simulink model "heli_q8_lab4_2020b"  (R2020b)
settings: Solver=ode1  StartTime=0.0  StopTime=inf  FixedStep=0.002  RelTol=1e-3  EnableMultiTasking=on
PostLoadFcn:
  | qc_set_target_type(getConfigSet(bdroot, 'QUARC Default Target Configuration'));
values from neighbouring files (symbols this model uses):
  Ad = sysd.A    [init_heli_3_10_part_4.m]    (also in tune_qw_offline.m = sd.A)
  Bd = sysd.B    [init_heli_3_10_part_4.m]    (also in tune_qw_offline.m = sd.B)
  Cd = sysd.C    [init_heli_3_10_part_4.m]    (also in tune_qw_offline.m = sd.C)
  elev_const = 0.53    [init_heli_3_10_part_4.m]
  F_2 = [K_2(1,1) K_2(1,3) ... (first row only)    [init_heli_3_10_part_4.m]
  gyro_bias = [0.0392850152533 -0.00867648252983 0.000660862987064]    [imu_bias.mat]    (also in update_imu_bias.m = mean(d(idx,13:15))')
  imu_bias = [-0.0918732538603 0 0.0496947738021 0 0]    [imu_bias.mat]    (also in update_imu_bias.m = imu_bias + mean(d(idx,2:6) - d(idx,8:12))')
  Joystick_gain_x = 1    [init_heli_3_10_part_4.m]
  Joystick_gain_y = -1    [init_heli_3_10_part_4.m]
  K_2 = lqr(A_lqr,B_lqr,Q_lqr, R_lqr)    [init_heli_3_10_part_4.m]
  P0 = blkdiag(P0, 0.02^2*eye(3))    [init_heli_3_10_part_4.m]
  Qd = Qd6    [init_heli_3_10_part_4.m]    (also in tune_qw_offline.m = blkdiag(Qd, 1e-11*eye(3)))
  Rd = [0.000112260066924 4.65584239908e-05 -7.15809020323e-05 -6.37518998984e-05 -2.81466202083e-06 4.65584239908e-05 0.000458002814453 2.17937662307e-05 -6.23292915171e-05 -4.71096272763e-06 -7.15809020323e-05 2.17937662307e-05 ... (25 elements, 5x5)]    [Rd.mat]    (also in analyze_noise.m = Rd_fly; estimate_Rd.m = cov(noise))
  V_s_0 = 7.77    [init_heli_3_10_part_4.m]
  x0 = [x0; 0; 0; 0]    [init_heli_3_10_part_4.m]
undefined symbols (not defined in the file or in its folder): HIL, qc_get_step_size, sigbuilder_block
libraries: quarc_library x9
settings Model: SimulationMode=external  ExtModeTrigDuration=50000  Creator=Rchan  LastModifiedBy=saavim
settings SolverCC: PositivePriorityOrder=on
settings DataIOCC: LimitDataPoints=on  SaveFormat=Array  SignalLoggingSaveFormat=ModelDataLogs  ReturnWorkspaceOutputs=off
settings OptimizationCC: ExpressionDepthLimit=2147483647  InitFltsAndDblsToZero=on  LifeSpan=inf
settings DebuggingCC: SaveWithParameterizedLinksMsg=none  UnderspecifiedInitializationDetection=Classic  MergeDetectMultiDrivingBlocksExec=none  SolverPrmCheckMsg=warning  MultiTaskDSMMsg=warning  MultiTaskCondExecSysMsg=none  FcnCallInpInsideContextMsg=warning  AllowSymbolicDim=off  StateNameClashWarn=warning  SFUnexpectedBacktrackingDiag=warning  SFNoUnconditionalDefaultTransitionDiag=warning  SFExecutionAtInitializationDiag=none  ArithmeticOperatorsInVariantConditions=warning
settings HardwareCC: ProdBitPerPointer=32  ProdBitPerSizeT=32  ProdBitPerPtrDiffT=32  ProdLargestAtomicFloat=None  ProdIntDivRoundTo=Undefined  ProdEndianess=Unspecified  ProdWordSize=32  ProdHWDeviceType=32-bit Generic
settings ModelReferenceCC: PropagateSignalLabelsOutOfModel=off
settings SFSimCC: SimUseLocalCustomCode=off  CustomCodeUndefinedFunction=UseInterfaceOnly
settings RTWCC: Description=QUARC Win64 Target  SystemTargetFile=quarc_win64.tlc  TemplateMakefile=quarc_default_tmf  RTWUseLocalCustomCode=off
settings CodeAppCC: StateflowObjectComments=on
settings STFCustomTargetCC: MatFileLogging=on
settings GRTTargetCC: TargetLangStandard=C89/C90 (ANSI)  ParMdlRefBuildCompliant=off  CompOptLevelCompliant=off  CombineOutputUpdateFcns=off  GRTInterface=on  UseToolchainInfoCompliant=off  ExtMode=on  ExtModeMexFile=quarc_comm
settings ConfigComp: CovMetricSettings=de  CovSaveCumulativeToWorkspaceVar=on  CovSaveSingleToWorkspaceVar=on  CovExternalEMLEnable=off  CovSFcnEnable=off

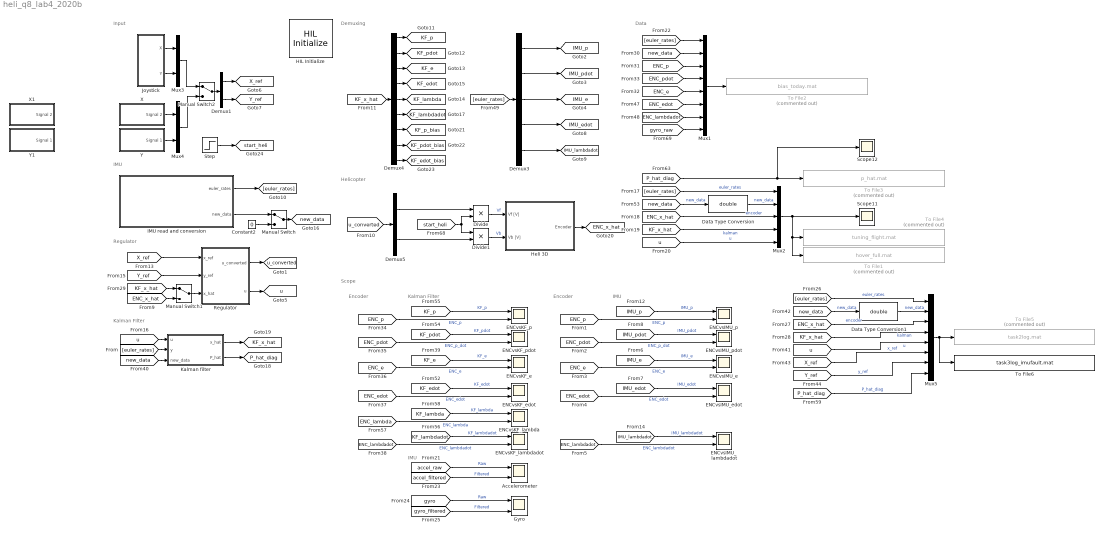
== system heli_q8_lab4_2020b ==
  note: Data
  note: Scope
  note: Helicopter
  note: Regulator
  note: IMU
  note: Kalman FIlter
  note: Input
  note: Demuxing
  note: Encoder
  note: Kalman Filter
  note: IMU
  note: Encoder
  note: IMU
  Accelerometer : Scope  NumInputPorts=2
  Constant2 : Constant  Value=0
  Data Type Conversion : DataTypeConversion  OutDataTypeStr=double  LockScale=on
  Data Type Conversion1 : DataTypeConversion  OutDataTypeStr=double  LockScale=on
  Demux1 : Demux  Outputs=2
  Demux3 : Demux  Outputs=5
  Demux4 : Demux  Outputs=9
  Demux5 : Demux  Outputs=2
  Divide : Product  Inputs=**
  Divide1 : Product  Inputs=**
  ENCvsIMU_e : Scope  NumInputPorts=2
  ENCvsIMU_edot : Scope  NumInputPorts=2
  ENCvsIMU_lambdadot : Scope  NumInputPorts=2
  ENCvsIMU_p : Scope  NumInputPorts=2
  ENCvsIMU_pdot : Scope  NumInputPorts=2
  ENCvsKF_e : Scope  NumInputPorts=2
  ENCvsKF_edot : Scope  NumInputPorts=2
  ENCvsKF_lambda : Scope  NumInputPorts=2
  ENCvsKF_lambdadot : Scope  NumInputPorts=2
  ENCvsKF_p : Scope  NumInputPorts=2
  ENCvsKF_pdot : Scope  NumInputPorts=2
  Gyro : Scope  NumInputPorts=2
  HIL Initialize : quarc_library/Data Acquisition/Generic/Configuration/HIL Initialize  Priority=-99  object_name=HIL-1  board_type=q8_usb  board_number=0  board_options=update_rate=normal;decimation=1  exclusive=off  active=off  hardware_clocks=[0:2]  clock_modes=[]  initial_clock_frequencies=[]  set_clock_params_at_start=off  set_clock_params_at_switch_in=off  set_clock_frequencies_at_start=off  set_clock_frequencies_at_switch_in=off  analog_input_channels=[0:7]  analog_input_configurations=[]  analog_input_maximums=10  analog_input_minimums=-10  set_analog_input_params_at_start=on  set_analog_input_params_at_switch_in=off  analog_output_channels=[0:7]  analog_output_maximums=10  analog_output_minimums=-10  initial_analog_outputs=[0]  final_analog_outputs=[0]  watchdog_analog_outputs=0  set_analog_output_params_at_start=on  set_analog_output_params_at_switch_in=off  set_analog_outputs_at_start=on  set_analog_outputs_at_switch_in=off  set_analog_outputs_at_terminate=on  set_analog_outputs_at_switch_out=off  set_analog_outputs_on_watchdog=off  digital_input_channels=[]  digital_output_channels=[]  digital_output_configuration=[]  initial_digital_outputs=[1]  final_digital_outputs=[1]  watchdog_digital_outputs=[1]  set_digital_output_params_at_start=off  set_digital_output_params_at_switch_in=off  set_digital_outputs_at_start=on  set_digital_outputs_at_switch_in=off  set_digital_outputs_at_terminate=on  set_digital_outputs_at_switch_out=off  set_digital_outputs_on_watchdog=off  encoder_channels=[0:7]  quadrature=[4]  encoder_filter_frequency=[]  initial_encoder_counts=[0]  set_encoder_params_at_start=on  set_encoder_params_at_switch_in=off  set_encoder_counts_at_start=on  set_encoder_counts_at_switch_in=off  pwm_channels=[0:7]  pwm_modes=0  pwm_frequency=99.532799999999995e6/4095  pwm_configuration=[0]  pwm_alignment=[0]  pwm_polarity=[1]  pwm_leading_deadband=[0]  pwm_trailing_deadband=[0]  initial_pwm_outputs=[0]  final_pwm_outputs=[0]  watchdog_pwm_outputs=[0]  set_pwm_params_at_start=on  set_pwm_params_at_switch_in=off  set_pwm_outputs_at_start=on  set_pwm_outputs_at_switch_in=off  set_pwm_outputs_at_terminate=on  set_pwm_outputs_at_switch_out=off  set_pwm_outputs_on_watchdog=off  other_output_channels=[]  initial_other_outputs=[]  final_other_outputs=[]  watchdog_other_outputs=[]  set_other_outputs_at_start=off  set_other_outputs_at_switch_in=off  set_other_outputs_at_terminate=off  set_other_outputs_at_switch_out=off  set_other_outputs_on_watchdog=off
  Heli 3D : Subsystem
  IMU read and conversion : Subsystem
  Joystick : Subsystem
  Kalman filter : Subsystem
  Manual Switch : ManualSwitch
  Manual Switch1 : ManualSwitch
  Manual Switch2 : ManualSwitch
  Mux1 : Mux  Inputs=8
  Mux2 : Mux  Inputs=5
  Mux3 : Mux  Inputs=2
  Mux4 : Mux  Inputs=2
  Mux5 : Mux  Inputs=8
  Regulator : Subsystem
  Scope11 : Scope
  Scope12 : Scope
  Step : Step  Time=3  SampleTime=0
  To File1 : ToFile  Commented=on  Filename=hover_full.mat  MatrixName=hover_full  SampleTime=0.002
  To File2 : ToFile  Commented=on  Filename=bias_today.mat  MatrixName=bias_today
  To File3 : ToFile  Commented=on  Filename=p_hat.mat  MatrixName=p_hat  SampleTime=0.002
  To File4 : ToFile  Commented=on  Filename=tuning_flight.mat  MatrixName=tuning_flight  SampleTime=0.002
  To File5 : ToFile  Commented=on  Filename=task2log.mat  MatrixName=task2log  SampleTime=0.002
  To File6 : ToFile  Filename=task3log_imufault.mat  MatrixName=task3log_imufault  SampleTime=0.002
  X : Subsystem  Tag=STV Subsys  LoadFcn=sigbuilder_block('load');  StartFcn=sigbuilder_block('start');  StopFcn=sigbuilder_block('stop');  ClipboardFcn=sigbuilder_block('clipboard');  mask(Sigbuilder block){tuvar=[0:10]}
      mask help: Simulink:masks:SigbuilderBlock_MD
      mask init:
      | if ~strcmp(get_param(bdroot(gcbh),'SimulationStatus'),'stopped') tuvar = sigbuilder_block('maskInit'); end
      settings: CopyFcn=sigbuilder_block('copy');  DeleteFcn=sigbuilder_block('delete');  ModelCloseFcn=sigbuilder_block('modelClose');  PreSaveFcn=sigbuilder_block('preSave');  PauseFcn=sigbuilder_block('pause');  ContinueFcn=sigbuilder_block('continue');  NameChangeFcn=sigbuilder_block('namechange');  OpenFcn=sigbuilder_block('open',[0 172 1440 619 ]);  CloseFcn=sigbuilder_block('close');
      mask Display: plot(0, 0, 100, 100,[2, 2, 32, 32, 2], [68, 8, 8, 68, 68],[32, 2], [38, 38], [32, 19, 2],[53, 60, 44], [32, 17, 17, 2],[16, 16, 31, 31]);txt = getActiveGroup(gcbh);text(2, 100, txt,'verticalAlignment', 'top');
  X1 : Subsystem  Tag=STV Subsys  LoadFcn=sigbuilder_block('load');  StartFcn=sigbuilder_block('start');  StopFcn=sigbuilder_block('stop');  ClipboardFcn=sigbuilder_block('clipboard');  mask(Sigbuilder block){tuvar=[0:10]}
      mask help: Simulink:masks:SigbuilderBlock_MD
      mask init:
      | if ~strcmp(get_param(bdroot(gcbh),'SimulationStatus'),'stopped') tuvar = sigbuilder_block('maskInit'); end
      settings: CopyFcn=sigbuilder_block('copy');  DeleteFcn=sigbuilder_block('delete');  ModelCloseFcn=sigbuilder_block('modelClose');  PreSaveFcn=sigbuilder_block('preSave');  PauseFcn=sigbuilder_block('pause');  ContinueFcn=sigbuilder_block('continue');  NameChangeFcn=sigbuilder_block('namechange');  OpenFcn=sigbuilder_block('open',[0 172 1440 619 ]);  CloseFcn=sigbuilder_block('close');
      mask Display: plot(0, 0, 100, 100,[2, 2, 32, 32, 2], [68, 8, 8, 68, 68],[32, 2], [38, 38], [32, 19, 2],[53, 60, 44], [32, 17, 17, 2],[16, 16, 31, 31]);txt = getActiveGroup(gcbh);text(2, 100, txt,'verticalAlignment', 'top');
  Y : Subsystem  Tag=STV Subsys  LoadFcn=sigbuilder_block('load');  StartFcn=sigbuilder_block('start');  StopFcn=sigbuilder_block('stop');  ClipboardFcn=sigbuilder_block('clipboard');  mask(Sigbuilder block){tuvar=[0:10]}
      mask help: Simulink:masks:SigbuilderBlock_MD
      mask init:
      | if ~strcmp(get_param(bdroot(gcbh),'SimulationStatus'),'stopped') tuvar = sigbuilder_block('maskInit'); end
      settings: CopyFcn=sigbuilder_block('copy');  DeleteFcn=sigbuilder_block('delete');  ModelCloseFcn=sigbuilder_block('modelClose');  PreSaveFcn=sigbuilder_block('preSave');  PauseFcn=sigbuilder_block('pause');  ContinueFcn=sigbuilder_block('continue');  NameChangeFcn=sigbuilder_block('namechange');  OpenFcn=sigbuilder_block('open',[217.5 306 1336.5 574.5 ]);  CloseFcn=sigbuilder_block('close');
      mask Display: plot(0, 0, 100, 100,[2, 2, 32, 32, 2], [68, 8, 8, 68, 68],[32, 2], [38, 38], [32, 19, 2],[53, 60, 44], [32, 17, 17, 2],[16, 16, 31, 31]);txt = getActiveGroup(gcbh);text(2, 100, txt,'verticalAlignment', 'top');
  Y1 : Subsystem  Tag=STV Subsys  LoadFcn=sigbuilder_block('load');  StartFcn=sigbuilder_block('start');  StopFcn=sigbuilder_block('stop');  ClipboardFcn=sigbuilder_block('clipboard');  mask(Sigbuilder block){tuvar=[0:10]}
      mask help: Simulink:masks:SigbuilderBlock_MD
      mask init:
      | if ~strcmp(get_param(bdroot(gcbh),'SimulationStatus'),'stopped') tuvar = sigbuilder_block('maskInit'); end
      settings: CopyFcn=sigbuilder_block('copy');  DeleteFcn=sigbuilder_block('delete');  ModelCloseFcn=sigbuilder_block('modelClose');  PreSaveFcn=sigbuilder_block('preSave');  PauseFcn=sigbuilder_block('pause');  ContinueFcn=sigbuilder_block('continue');  NameChangeFcn=sigbuilder_block('namechange');  OpenFcn=sigbuilder_block('open',[217.5 306 1336.5 574.5 ]);  CloseFcn=sigbuilder_block('close');
      mask Display: plot(0, 0, 100, 100,[2, 2, 32, 32, 2], [68, 8, 8, 68, 68],[32, 2], [38, 38], [32, 19, 2],[53, 60, 44], [32, 17, 17, 2],[16, 16, 31, 31]);txt = getActiveGroup(gcbh);text(2, 100, txt,'verticalAlignment', 'top');
  tag scope: ENC_x_hat=global, IMU_e=global, IMU_edot=global, IMU_lambdadot=global, IMU_p=global, IMU_pdot=global, KF_e=global, KF_edot=global, KF_edot_bias=global, KF_lambda=global, KF_lambdadot=global, KF_p=global, KF_p_bias=global, KF_pdot=global, KF_pdot_bias=global, KF_x_hat=global, P_hat_diag=global, X_ref=global, Y_ref=global, new_data=global, start_heli=global, u=global, u_converted=global
  wires:
  IMU read and conversion/1(euler_rates) -> [euler_rates]
  Kalman filter/1(x_hat) -> [KF_x_hat]
  Demux4/1 -> [KF_p]
  Demux4/2 -> [KF_pdot]
  Demux4/3 -> [KF_e]
  Demux4/4 -> [KF_edot]
  Demux4/5 -> [KF_lambda]
  [new_data] -> Kalman filter/3(new_data)
  [euler_rates] -> Kalman filter/2(y)
  [new_data] -> Data Type Conversion/1  "new_data"
  Demux4/6 -> [KF_lambdadot]
  Kalman filter/2(P_hat) -> [P_hat_diag]
  Mux2/1 -> To File4/1, To File1/1, Scope11/1
  [P_hat_diag] -> Scope12/1, To File3/1
  IMU read and conversion/2(new_data) -> Manual Switch/1
  Manual Switch/1 -> [new_data]
  Constant2/1 -> Manual Switch/2
  Mux1/1 -> To File2/1
  [euler_rates] -> Mux1/1
  [new_data] -> Mux1/2
  [ENC_p] -> Mux1/3
  [ENC_pdot] -> Mux1/4
  [ENC_e] -> Mux1/5
  [ENC_edot] -> Mux1/6
  [ENC_lambdadot] -> Mux1/7
  [euler_rates] -> Demux3/1
  Demux4/7 -> [KF_p_bias]
  Demux4/8 -> [KF_pdot_bias]
  Demux4/9 -> [KF_edot_bias]
  Step/1 -> [start_heli]
  [start_heli] -> Divide/2, Divide1/1
  [gyro_raw] -> Mux1/8
  Divide/1 -> Heli 3D/1(Vf [V])  "Vf"
  Divide1/1 -> Heli 3D/2(Vb [V])  "Vb"
  Heli 3D/1(Encoder) -> [ENC_x_hat]
  Demux5/2 -> Divide1/2
  Demux5/1 -> Divide/1
  [u_converted] -> Demux5/1
  [KF_x_hat] -> Demux4/1
  [KF_x_hat] -> Manual Switch1/1
  [ENC_x_hat] -> Manual Switch1/2
  Demux3/1 -> [IMU_p]
  Demux3/2 -> [IMU_pdot]
  Demux3/3 -> [IMU_e]
  Demux3/4 -> [IMU_edot]
  Demux3/5 -> [IMU_lambdadot]
  Manual Switch2/1 -> Demux1/1
  Demux1/1 -> [X_ref]
  Demux1/2 -> [Y_ref]
  Joystick/1(X) -> Mux3/1
  Joystick/2(Y) -> Mux3/2
  Mux3/1 -> Manual Switch2/1
  X/1(Signal 2) -> Mux4/1
  Y/1(Signal 1) -> Mux4/2
  Mux4/1 -> Manual Switch2/2
  [X_ref] -> Regulator/1(x_ref)
  [Y_ref] -> Regulator/2(y_ref)
  Manual Switch1/1 -> Regulator/3(x_hat)
  Regulator/1(u_converted) -> [u_converted]
  Regulator/2(u) -> [u]
  [euler_rates] -> Mux2/1  "euler_rates"
  Data Type Conversion/1 -> Mux2/2  "new_data"
  [ENC_x_hat] -> Mux2/3  "encoder"
  [KF_x_hat] -> Mux2/4  "kalman"
  [u] -> Mux2/5  "u"
  [u] -> Kalman filter/1(u)
  [IMU_p] -> ENCvsIMU_p/1  "IMU_p"
  [ENC_p] -> ENCvsIMU_p/2  "ENC_p"
  [IMU_pdot] -> ENCvsIMU_pdot/1  "IMU_pdot"
  [ENC_pdot] -> ENCvsIMU_pdot/2  "ENC_p_dot"
  [IMU_e] -> ENCvsIMU_e/1  "IMU_e"
  [ENC_e] -> ENCvsIMU_e/2  "ENC_e"
  [IMU_edot] -> ENCvsIMU_edot/1  "IMU_edot"
  [ENC_edot] -> ENCvsIMU_edot/2  "ENC_edot"
  [IMU_lambdadot] -> ENCvsIMU_lambdadot/1  "IMU_lambdadot"
  [ENC_lambdadot] -> ENCvsIMU_lambdadot/2  "ENC_lambdadot"
  [ENC_p] -> ENCvsKF_p/2  "ENC_p"
  [KF_p] -> ENCvsKF_p/1  "KF_p"
  [KF_pdot] -> ENCvsKF_pdot/1  "KF_pdot"
  [ENC_pdot] -> ENCvsKF_pdot/2  "ENC_p_dot"
  [KF_e] -> ENCvsKF_e/1  "KF_e"
  [ENC_e] -> ENCvsKF_e/2  "ENC_e"
  [KF_edot] -> ENCvsKF_edot/1  "KF_edot"
  [ENC_edot] -> ENCvsKF_edot/2  "ENC_edot"
  [KF_lambda] -> ENCvsKF_lambda/1  "KF_lambda"
  [ENC_lambda] -> ENCvsKF_lambda/2  "ENC_lambda"
  [KF_lambdadot] -> ENCvsKF_lambdadot/1  "KF_lambdadot"
  [ENC_lambdadot] -> ENCvsKF_lambdadot/2  "ENC_lambdadot"
  [accel_raw] -> Accelerometer/1  "Raw"
  [accel_filtered] -> Accelerometer/2  "Filtered"
  [gyro] -> Gyro/1  "Raw"
  [gyro_filtered] -> Gyro/2  "Filtered"
  Mux5/1 -> To File6/1, To File5/1
  [euler_rates] -> Mux5/1  "euler_rates"
  [new_data] -> Data Type Conversion1/1  "new_data"
  Data Type Conversion1/1 -> Mux5/2  "new_data"
  [ENC_x_hat] -> Mux5/3  "encoder"
  [KF_x_hat] -> Mux5/4  "kalman"
  [u] -> Mux5/5  "u"
  [X_ref] -> Mux5/6  "x_ref"
  [Y_ref] -> Mux5/7  "y_ref"
  [P_hat_diag] -> Mux5/8  "P_hat_diag"

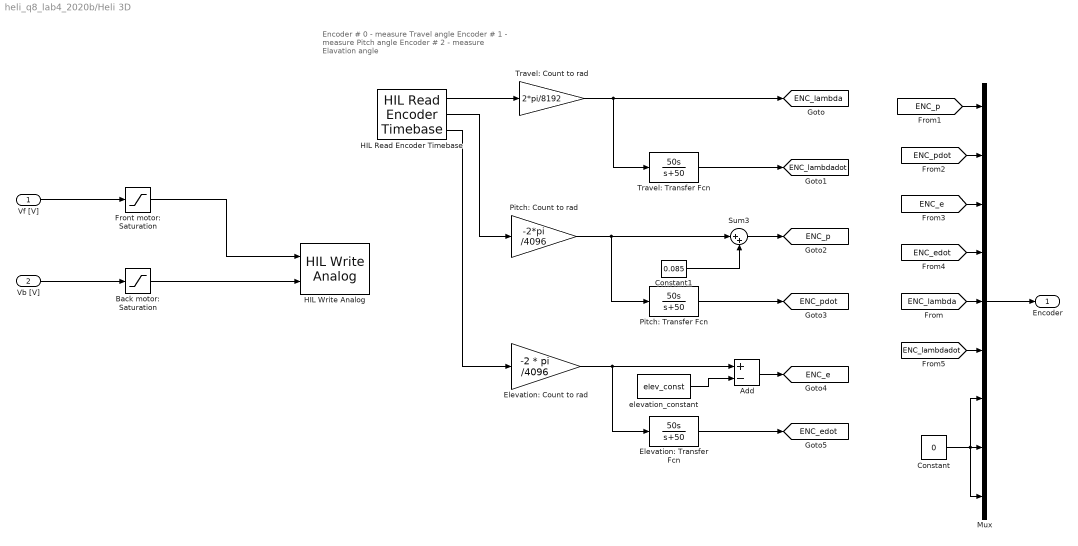
== system heli_q8_lab4_2020b/Heli 3D ==
  note: Encoder # 0 - measure Travel angle
      | Encoder # 1 - measure Pitch angle
      | Encoder # 2 - measure Elavation angle
  Vf [V] : Inport
  Vb [V] : Inport  Port=2
  Add : Sum  Inputs=+-
  Back motor: Saturation : Saturate  UpperLimit=5  LowerLimit=-5
  Constant : Constant  Value=0
  Constant1 : Constant  Value=0.085
  Elevation: Count to rad : Gain  Gain=-2 * pi /4096
  Elevation: Transfer Fcn : TransferFcn  Numerator=[50 0]  Denominator=[1 50]
  Front motor: Saturation : Saturate  UpperLimit=5  LowerLimit=-5
  HIL Read Encoder Timebase : quarc_library/Data Acquisition/Generic/Timebases/HIL Read Encoder Timebase  object_name=HIL-1  clock=0  channels=[0:2]  active=on  vector_output=off  data_type_mode=Inherit via back propagation  data_type=double  overflow_mode=Error on overflow  samples_in_buffer=max(ceil(1/qc_get_step_size), 1)
  HIL Write Analog : quarc_library/Data Acquisition/Generic/Immediate I//O/HIL Write Analog  object_name=HIL-1  channels=[0:1]  sample_time=-1  active=off  vector_input=off
  Mux : Mux  Inputs=9
  Pitch: Count to rad : Gain  Gain=-2*pi /4096
  Pitch: Transfer Fcn : TransferFcn  Numerator=[50 0]  Denominator=[1 50]
  Sum3 : Sum  Inputs=|++
  Travel: Count to rad : Gain  Gain=2*pi/8192
  Travel: Transfer Fcn : TransferFcn  Numerator=[50 0]  Denominator=[1 50]
  elevation_constant : Constant  Value=elev_const
  Encoder : Outport
  tag scope: ENC_e=global, ENC_edot=global, ENC_lambda=global, ENC_lambdadot=global, ENC_p=global, ENC_pdot=global
  wires:
  HIL Read Encoder Timebase/1 -> Travel: Count to rad/1
  HIL Read Encoder Timebase/2 -> Pitch: Count to rad/1
  HIL Read Encoder Timebase/3 -> Elevation: Count to rad/1
  Travel: Count to rad/1 -> Travel: Transfer Fcn/1, [ENC_lambda]
  Travel: Transfer Fcn/1 -> [ENC_lambdadot]
  Elevation: Count to rad/1 -> Add/1, Elevation: Transfer Fcn/1
  Elevation: Transfer Fcn/1 -> [ENC_edot]
  Vf [V]/1 -> Front motor: Saturation/1
  Vb [V]/1 -> Back motor: Saturation/1
  Front motor: Saturation/1 -> HIL Write Analog/1
  Back motor: Saturation/1 -> HIL Write Analog/2
  elevation_constant/1 -> Add/2
  Add/1 -> [ENC_e]
  Pitch: Count to rad/1 -> Pitch: Transfer Fcn/1, Sum3/1
  Pitch: Transfer Fcn/1 -> [ENC_pdot]
  Constant1/1 -> Sum3/2
  Sum3/1 -> [ENC_p]
  Mux/1 -> Encoder/1
  [ENC_p] -> Mux/1
  [ENC_pdot] -> Mux/2
  Constant/1 -> Mux/9, Mux/7, Mux/8
  [ENC_lambdadot] -> Mux/6
  [ENC_lambda] -> Mux/5
  [ENC_edot] -> Mux/4
  [ENC_e] -> Mux/3

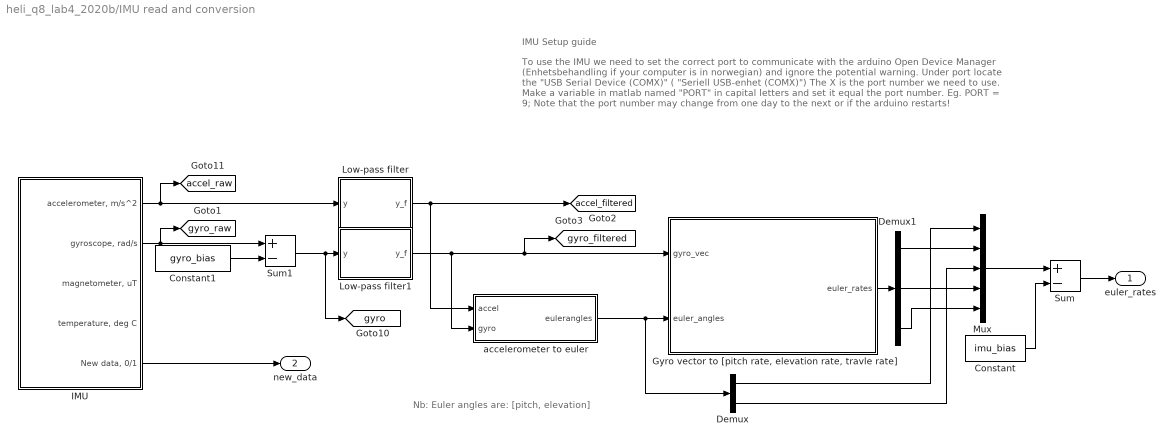
== system heli_q8_lab4_2020b/IMU read and conversion ==
  note: Nb: Euler angles are: [pitch, elevation]
  note: IMU Setup guide
  note: To use the IMU we need to set the correct port to communicate with the arduino
      | Open Device Manager (Enhetsbehandling if your computer is in norwegian) and ignore the potential warning.
      | Under port locate the "USB Serial Device (COMX)" ( "Seriell USB-enhet (COMX)")
      | The X is the port number we need to use.
      |
      | Make a variable in matlab named "PORT" in capital letters and set it equal the port number.
      | Eg.
      | PORT = 9;
      |
      | Note that the port number may change from one day to the next or if the arduino restarts!
  Constant : Constant  Value=imu_bias
  Constant1 : Constant  Value=gyro_bias
  Demux : Demux  Outputs=2
  Demux1 : Demux  Outputs=3
  "Gyro vector to [pitch rate, elevation rate, travle rate]" : MATLAB Function  TreatAsAtomicUnit=on
  IMU : Subsystem
  Low-pass filter : MATLAB Function  TreatAsAtomicUnit=on
  Low-pass filter1 : MATLAB Function  TreatAsAtomicUnit=on
  Mux : Mux  Inputs=5
  Sum : Sum  Inputs=+-
  Sum1 : Sum  Inputs=+-
  accelerometer to euler : MATLAB Function  TreatAsAtomicUnit=on
  euler_rates : Outport
  new_data : Outport  Port=2
  tag scope: accel_filtered=global, accel_raw=global, gyro=global, gyro_filtered=global, gyro_raw=global
  wires:
  IMU/2("gyroscope, rad/s") -> Sum1/1, [gyro_raw]
  "Gyro vector to [pitch rate, elevation rate, travle rate]"/1(euler_rates) -> Demux1/1
  Demux/1 -> Mux/1
  Demux1/1 -> Mux/2
  Demux/2 -> Mux/3
  Demux1/2 -> Mux/4
  Demux1/3 -> Mux/5
  IMU/5("New data, 0/1") -> new_data/1
  IMU/1("accelerometer, m/s^2") -> [accel_raw], Low-pass filter/1(y)
  accelerometer to euler/1(eulerangles) -> Demux/1, "Gyro vector to [pitch rate, elevation rate, travle rate]"/2(euler_angles)
  Constant/1 -> Sum/2
  Constant1/1 -> Sum1/2
  Sum1/1 -> [gyro], Low-pass filter1/1(y)
  Sum/1 -> euler_rates/1
  Mux/1 -> Sum/1
  Low-pass filter/1(y_f) -> [accel_filtered], accelerometer to euler/1(accel)
  Low-pass filter1/1(y_f) -> [gyro_filtered], "Gyro vector to [pitch rate, elevation rate, travle rate]"/1(gyro_vec), accelerometer to euler/2(gyro)

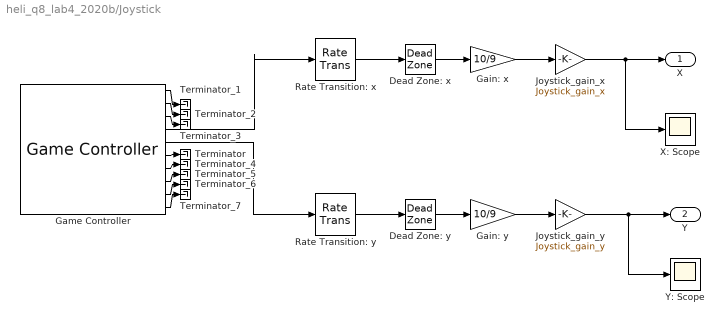
== system heli_q8_lab4_2020b/Joystick ==
  Dead Zone: x : DeadZone  LowerValue=-0.1  UpperValue=0.1  SaturateOnIntegerOverflow=on
  Dead Zone: y : DeadZone  LowerValue=-0.1  UpperValue=0.1  SaturateOnIntegerOverflow=on
  Gain: x : Gain  Gain=10/9
  Gain: y : Gain  Gain=10/9
  Game Controller : quarc_library/Devices/Peripherals/Target/Game Controller  controller=1  buffer_size=12  deadzone=[]  saturation=[]  sample_time=max(qc_get_step_size, 0.01)  auto_center=off  enabled=on
      settings: SourceProductName=QUARC Targets
  Joystick_gain_x : Gain  Gain=Joystick_gain_x
  Joystick_gain_y : Gain  Gain=Joystick_gain_y
  Rate Transition: x : RateTransition
  Rate Transition: y : RateTransition
  Terminator : Terminator
  Terminator_{1..7} (7 alike) : Terminator
  X: Scope : Scope
  Y: Scope : Scope
  X : Outport
  Y : Outport  Port=2
  wires:
  Rate Transition: y/1 -> Dead Zone: y/1
  Rate Transition: x/1 -> Dead Zone: x/1
  Game Controller/5 -> Rate Transition: y/1
  Game Controller/4 -> Rate Transition: x/1
  Game Controller/1 -> Terminator_1/1
  Game Controller/2 -> Terminator_2/1
  Game Controller/7 -> Terminator_4/1
  Game Controller/8 -> Terminator_5/1
  Game Controller/9 -> Terminator_6/1
  Game Controller/10 -> Terminator_7/1
  Game Controller/6 -> Terminator/1
  Dead Zone: x/1 -> Gain: x/1
  Dead Zone: y/1 -> Gain: y/1
  Gain: x/1 -> Joystick_gain_x/1
  Gain: y/1 -> Joystick_gain_y/1
  Joystick_gain_x/1 -> X/1, X: Scope/1
  Joystick_gain_y/1 -> Y: Scope/1, Y/1
  Game Controller/3 -> Terminator_3/1

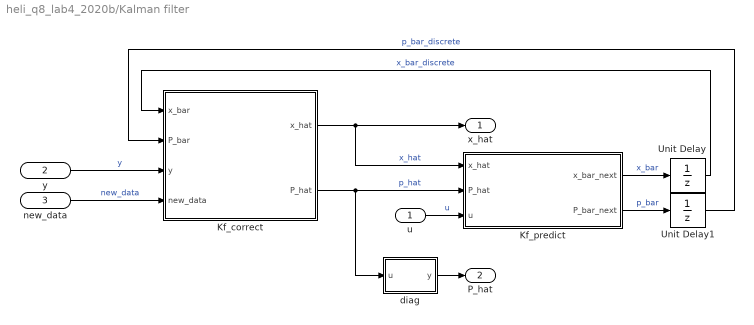
== system heli_q8_lab4_2020b/Kalman filter ==
  u : Inport
  y : Inport  Port=2
  new_data : Inport  Port=3
  Kf_correct : MATLAB Function  TreatAsAtomicUnit=on
  Kf_predict : MATLAB Function  TreatAsAtomicUnit=on
  Unit Delay : UnitDelay  InitialCondition=x0  SampleTime=0.002  HasFrameUpgradeWarning=on
  Unit Delay1 : UnitDelay  InitialCondition=P0  SampleTime=0.002  HasFrameUpgradeWarning=on
  diag : MATLAB Function  TreatAsAtomicUnit=on
  x_hat : Outport
  P_hat : Outport  Port=2
  wires:
  y/1 -> Kf_correct/3(y)  "y"
  Kf_predict/1(x_bar_next) -> Unit Delay/1  "x_bar"
  Kf_predict/2(P_bar_next) -> Unit Delay1/1  "p_bar"
  Kf_correct/1(x_hat) -> Kf_predict/1(x_hat), x_hat/1  "x_hat"
  Kf_correct/2(P_hat) -> diag/1(u), Kf_predict/2(P_hat)  "p_hat"
  u/1 -> Kf_predict/3(u)  "u"
  Unit Delay/1 -> Kf_correct/1(x_bar)  "x_bar_discrete"
  Unit Delay1/1 -> Kf_correct/2(P_bar)  "p_bar_discrete"
  new_data/1 -> Kf_correct/4(new_data)  "new_data"
  diag/1(y) -> P_hat/1

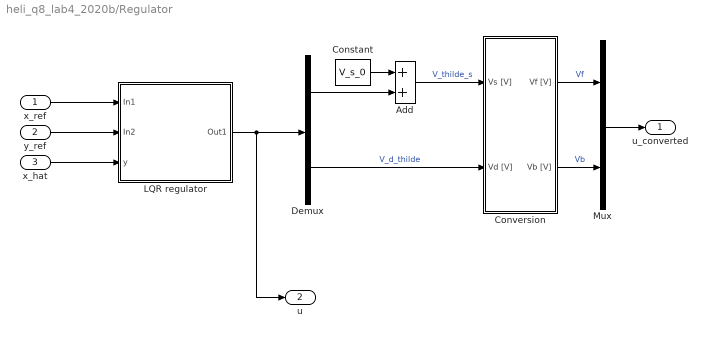
== system heli_q8_lab4_2020b/Regulator ==
  x_ref : Inport
  y_ref : Inport  Port=2
  x_hat : Inport  Port=3
  Add : Sum
  Constant : Constant  Value=V_s_0
  Conversion : Subsystem
  Demux : Demux  Outputs=2
  LQR regulator : Subsystem
  Mux : Mux  Inputs=2
  u_converted : Outport
  u : Outport  Port=2
  wires:
  Add/1 -> Conversion/1(Vs [V])  "V_thilde_s"
  Constant/1 -> Add/1
  Conversion/1(Vf [V]) -> Mux/1  "Vf"
  Demux/1 -> Add/2
  Conversion/2(Vb [V]) -> Mux/2  "Vb"
  x_ref/1 -> LQR regulator/1(In1)
  y_ref/1 -> LQR regulator/2(In2)
  LQR regulator/1(Out1) -> u/1, Demux/1
  Mux/1 -> u_converted/1
  x_hat/1 -> LQR regulator/3(y)
  Demux/2 -> Conversion/2(Vd [V])  "V_d_thilde"

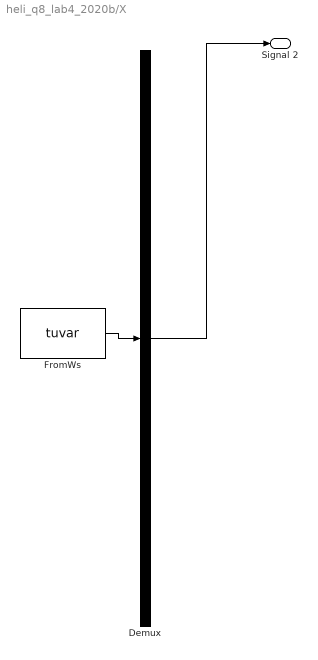
== system heli_q8_lab4_2020b/X ==
  Demux : Demux  Tag=STV Demux  Outputs=1
      settings: DisplayOption=none
  FromWs : FromWorkspace  Tag=STV FromWs  VariableName=tuvar
      SigBuilderData=|
      | common.afterFinalStr = 'Extrapolate'
      | common.sampleTime = 0
      | dataSet.timeRange = [0 90]
      | dataSet.name = 'Group 1'
      | sbobj.Groups.Name = 'Group 1'
      | sbobj.Groups.Signals.Name = 'Signal 2'
      | sbobj.Groups.Signals.XData = [0 35 35 40 40 45 45 50 50 55 55 60 60 70 70 75 75 90]
      | sbobj.Groups.Signals.YData = [0 0 0.3 0.3 0 0 -0.3 -0.3 0 0 0.5 0.5 0 0 -0.5 -0.5 0 0]
      | sbobj.Groups.TimeRange = [0 90]
  Signal 2 : Outport  Tag=STV Outport
  wires:
  Demux/1 -> Signal 2/1
  FromWs/1 -> Demux/1

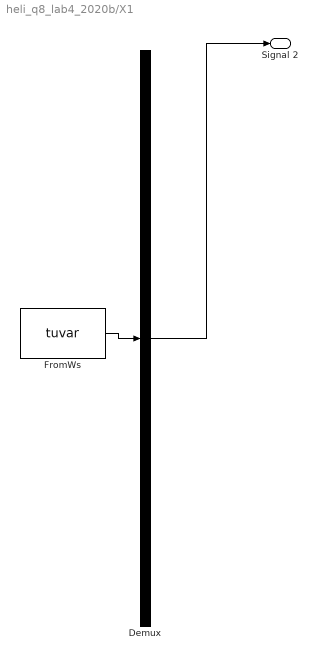
== system heli_q8_lab4_2020b/X1 ==
  Demux : Demux  Tag=STV Demux  Outputs=1
      settings: DisplayOption=none
  FromWs : FromWorkspace  Tag=STV FromWs  VariableName=tuvar
      SigBuilderData=|
      | common.afterFinalStr = 'Extrapolate'
      | common.sampleTime = 0
      | dataSet.timeRange = [0 60]
      | dataSet.name = 'Group 1'
      | sbobj.Groups.Name = 'Group 1'
      | sbobj.Groups.Signals.Name = 'Signal 2'
      | sbobj.Groups.Signals.XData = [0 10 10 15 15 30 30 35 35 60]
      | sbobj.Groups.Signals.YData = [0 0 0.4 0.4 0 0 -0.4 -0.4 0 0]
      | sbobj.Groups.TimeRange = [0 60]
  Signal 2 : Outport  Tag=STV Outport
  wires:
  Demux/1 -> Signal 2/1
  FromWs/1 -> Demux/1

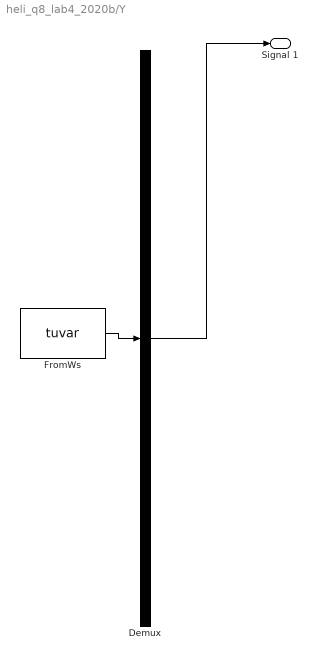
== system heli_q8_lab4_2020b/Y ==
  Demux : Demux  Tag=STV Demux  Outputs=1
      settings: DisplayOption=none
  FromWs : FromWorkspace  Tag=STV FromWs  VariableName=tuvar
      SigBuilderData=|
      | common.afterFinalStr = 'Extrapolate'
      | common.sampleTime = 0
      | dataSet.timeRange = [0 90]
      | dataSet.name = 'Group 1'
      | sbobj.Groups.Name = 'Group 1'
      | sbobj.Groups.Signals.Name = 'Signal 1'
      | sbobj.Groups.Signals.XData = [0 4 4 9.1 9.1 20 20 23 23 27 27 30 30 90]
      | sbobj.Groups.Signals.YData = [0 0 0.101 0.101 0 0 -0.2 -0.2 0 0 0.2 0.2 0 0]
      | sbobj.Groups.TimeRange = [0 90]
  Signal 1 : Outport  Tag=STV Outport
  wires:
  Demux/1 -> Signal 1/1
  FromWs/1 -> Demux/1

== system heli_q8_lab4_2020b/Y1 ==
  Demux : Demux  Tag=STV Demux  Outputs=1
      settings: DisplayOption=none
  FromWs : FromWorkspace  Tag=STV FromWs  VariableName=tuvar
      SigBuilderData=|
      | common.afterFinalStr = 'Extrapolate'
      | common.sampleTime = 0
      | dataSet.timeRange = [0 10]
      | dataSet.name = 'Group 1'
      | sbobj.Groups.Name = 'Group 1'
      | sbobj.Groups.Signals.Name = 'Signal 1'
      | sbobj.Groups.Signals.XData = [0 5.01 5.01 6 6 10]
      | sbobj.Groups.Signals.YData = [0 0 0.4 0.4 0 0]
  Signal 1 : Outport  Tag=STV Outport
  wires:
  Demux/1 -> Signal 1/1
  FromWs/1 -> Demux/1

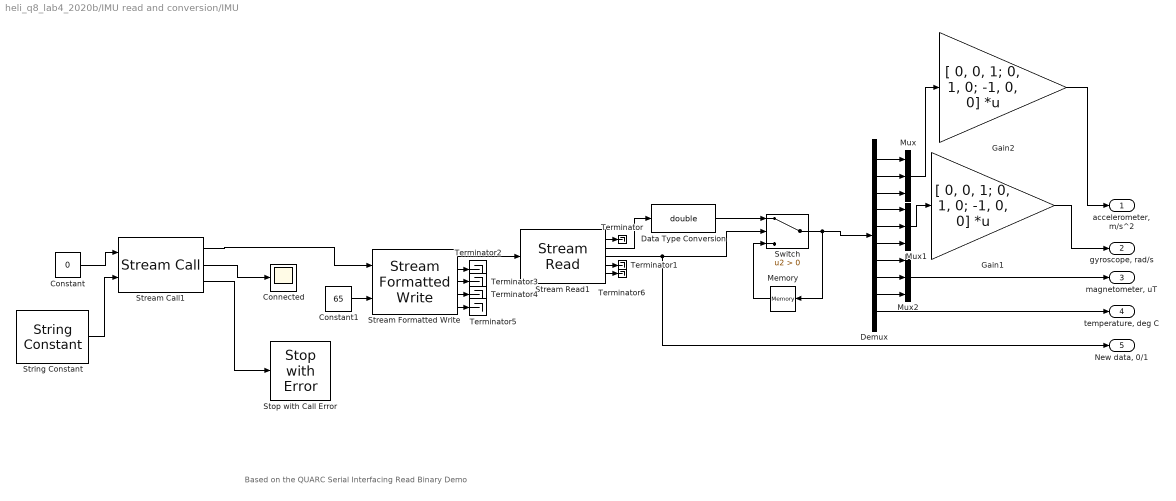
== system heli_q8_lab4_2020b/IMU read and conversion/IMU ==
  note: Based on the QUARC Serial Interfacing Read Binary Demo
  Connected : Scope
  Constant : Constant  Value=0
  Constant1 : Constant  Value=65
  Data Type Conversion : DataTypeConversion  OutDataTypeStr=double
  Demux : Demux  Outputs=10
  Gain1 : Gain  Gain=[ 0, 0, 1; 0, 1, 0; -1, 0, 0]  Multiplication=Matrix(K*u) (u vector)
  Gain2 : Gain  Gain=[ 0, 0, 1; 0, 1, 0; -1, 0, 0]  Multiplication=Matrix(K*u) (u vector)
  Memory : Memory  InitialCondition=[0 0 0 0 0 0 0 0 0 0]
  Mux : Mux  Inputs=3
  Mux1 : Mux  Inputs=3
  Mux2 : Mux  Inputs=3
  Stop with Call Error : quarc_library/Sinks/Error Handling/Stop with Error  message_type=Interpret input as error code  message=Error occurred
      settings: SourceProductName=QUARC Targets
  Stream Call1 : quarc_library/Communications/Intermediate/Stream Call  uri_source=External input port  uri=serial://IMU:9?baud=115200,word=8,parity=none,stop=1,flow='none'  apply_uri_to_all_configs=on  send_buffer_size=8000  receive_buffer_size=8000  byte_order=little endian (Intel - LSB first)  sample_time=qc_get_step_size  non_blocking=on  active=off
      settings: SourceProductName=QUARC Targets
  Stream Formatted Write : quarc_library/Communications/Intermediate/Stream Formatted Write  format_string=%c\n  max_code_units=80  optimization=Minimizing latency
      settings: SourceProductName=QUARC Targets
  Stream Read1 : quarc_library/Communications/Intermediate/Stream Read  data_type=single  type_expr=BusObject  num_elements=10  receive_dims=off
      settings: SourceProductName=QUARC Targets
  String Constant : quarc_library/Strings/String Constant  string_value=qc_perform_substitutions('serial://IMU:%{PORT}?baud=115200,word=8,parity=none,stop=1')  evaluate_string=on  string_type=URI  max_length=255  sample_time=inf  variable_size=off
      settings: AttributesFormatString="\"serial://IMU:6?baud=115200,word=8,parity=none,stop=1\""  SourceProductName=QUARC Targets
  Switch : Switch  Criteria=u2 > Threshold
  Terminator{,1..6} (7 alike) : Terminator
  "accelerometer, m/s^2" : Outport
  "gyroscope, rad/s" : Outport  Port=2
  "magnetometer, uT" : Outport  Port=3
  "temperature, deg C" : Outport  Port=4
  "New data, 0/1" : Outport  Port=5
  wires:
  Switch/1 -> Memory/1, Demux/1
  Data Type Conversion/1 -> Switch/1
  Stream Read1/3 -> "New data, 0/1"/1, Switch/2
  Stream Formatted Write/1 -> Stream Read1/1
  Constant1/1 -> Stream Formatted Write/2
  Gain1/1 -> "gyroscope, rad/s"/1
  Gain2/1 -> "accelerometer, m/s^2"/1
  Stream Read1/4 -> Terminator1/1
  Demux/10 -> "temperature, deg C"/1
  Mux1/1 -> Gain1/1
  Stream Read1/2 -> Data Type Conversion/1
  Demux/7 -> Mux2/1
  Demux/8 -> Mux2/2
  Demux/9 -> Mux2/3
  Mux2/1 -> "magnetometer, uT"/1
  Demux/6 -> Mux1/3
  Demux/5 -> Mux1/2
  Demux/4 -> Mux1/1
  Mux/1 -> Gain2/1
  Demux/3 -> Mux/3
  Demux/1 -> Mux/1
  Demux/2 -> Mux/2
  Stream Read1/1 -> Terminator/1
  Stream Call1/1 -> Stream Formatted Write/1
  Constant/1 -> Stream Call1/1
  String Constant/1 -> Stream Call1/2
  Stream Call1/2 -> Connected/1
  Stream Call1/3 -> Stop with Call Error/1
  Memory/1 -> Switch/3
  Stream Formatted Write/2 -> Terminator2/1
  Stream Formatted Write/3 -> Terminator3/1
  Stream Formatted Write/4 -> Terminator4/1
  Stream Formatted Write/5 -> Terminator5/1
  Stream Read1/5 -> Terminator6/1

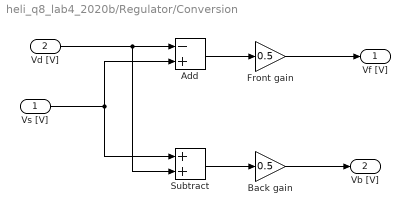
== system heli_q8_lab4_2020b/Regulator/Conversion ==
  Vs [V] : Inport
  Vd [V] : Inport  Port=2
  Add : Sum  Inputs=-+
  Back gain : Gain  Gain=0.5
  Front gain : Gain  Gain=0.5
  Subtract : Sum
  Vf [V] : Outport
  Vb [V] : Outport  Port=2
  wires:
  Vd [V]/1 -> Subtract/2, Add/1
  Vs [V]/1 -> Subtract/1, Add/2
  Subtract/1 -> Back gain/1
  Back gain/1 -> Vb [V]/1
  Add/1 -> Front gain/1
  Front gain/1 -> Vf [V]/1

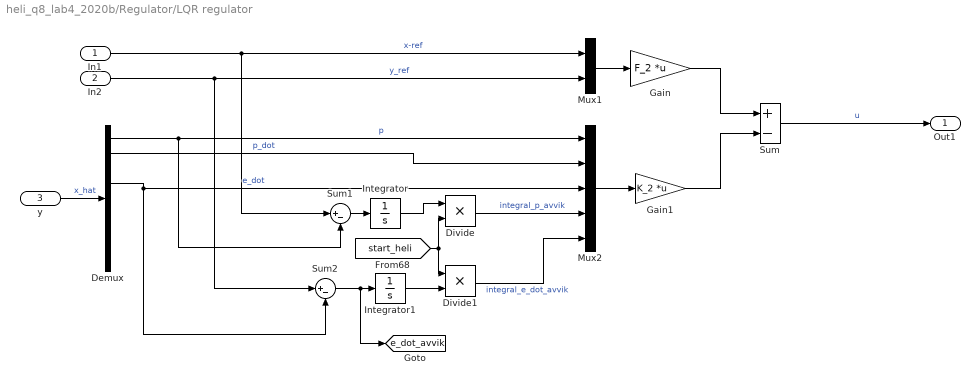
== system heli_q8_lab4_2020b/Regulator/LQR regulator ==
  In1 : Inport
  In2 : Inport  Port=2
  y : Inport  Port=3
  Demux : Demux  Outputs=9
  Divide : Product  Inputs=**
  Divide1 : Product  Inputs=**
  Gain : Gain  Gain=F_2  Multiplication=Matrix(K*u)
  Gain1 : Gain  Gain=K_2  Multiplication=Matrix(K*u)
  Integrator : Integrator
  Integrator1 : Integrator
  Mux1 : Mux  Inputs=2
  Mux2 : Mux  Inputs=5
  Sum : Sum  Inputs=+-
  Sum1 : Sum  Inputs=|+-
  Sum2 : Sum  Inputs=|+-
  Out1 : Outport
  tag scope: e_dot_avvik=global
  wires:
  Demux/1 -> Sum1/2, Mux2/1  "p"
  Integrator1/1 -> Divide1/2
  Demux/2 -> Mux2/2  "p_dot"
  Gain1/1 -> Sum/2
  Mux1/1 -> Gain/1
  Sum/1 -> Out1/1  "u"
  Mux2/1 -> Gain1/1
  Demux/4 -> Sum2/2, Mux2/3  "e_dot"
  Gain/1 -> Sum/1
  In1/1 -> Mux1/1, Sum1/1  "x-ref"
  In2/1 -> Mux1/2, Sum2/1  "y_ref"
  Sum1/1 -> Integrator/1
  Sum2/1 -> [e_dot_avvik], Integrator1/1
  y/1 -> Demux/1  "x_hat"
  Divide/1 -> Mux2/4  "integral_p_avvik"
  Integrator/1 -> Divide/1
  Divide1/1 -> Mux2/5  "integral_e_dot_avvik"
  [start_heli] -> Divide/2, Divide1/1

== matlab function heli_q8_lab4_2020b/IMU read and conversion/accelerometer to euler ==
  data: accel input; eulerangles output; gyro input
function eulerangles = fcn(accel, gyro)
l_h = 0.66; %Avstand elevasjonsakse - hode [m]
ax = accel(1);
ay = accel(2);
az = accel(3);

ax = ax + l_h*(gyro(2)^2 + gyro(3)^2); %Fjerner sentripetalaksellerasjonen

if abs(az) < 1e-3
    az = -1e-3;
end

pitch = atan(ay/az);
elevation = atan2(ax, sqrt(ay^2+az^2));

eulerangles = [pitch elevation];

== matlab function heli_q8_lab4_2020b/IMU read and conversion/Gyro vector to [pitch rate, elevation rate, travle rate] ==
  data: gyro_vec input; euler_rates output; euler_angles input
function euler_rates = gyro_vec_to_euler_rates(gyro_vec,euler_angles)
%#codegen
    phi = euler_angles(1);
    theta = euler_angles(2);
    %psi = euler_angles(3);


    T = [1, sin(phi)*tan(theta), cos(phi)*tan(theta);
         0, cos(phi),            -sin(phi);
         0, sin(phi)/cos(theta), cos(phi)/cos(theta)]; 
euler_rates = T*gyro_vec;

== matlab function heli_q8_lab4_2020b/Kalman filter/diag ==
  data: u input; y output
function y = fcn(u)
y = diag(u);

== matlab function heli_q8_lab4_2020b/Kalman filter/Kf_correct ==
  data: x_bar input; x_hat output; P_bar input; y input; new_data input; P_hat output; Cd parameter; Rd parameter
function [x_hat, P_hat] = kf_correct(x_bar, P_bar, y, new_data, Cd, Rd)
% Korrigerer kun når IMU har gitt en ny sample, ellers gir prediction
n = size(Cd, 2);
x_hat = zeros(n, 1);
P_hat = zeros(n, n);

if new_data > 0.5
    S = Cd*P_bar*Cd' + Rd;
    L = P_bar*Cd' / S;
    x_hat = x_bar + L*(y - Cd*x_bar);
    I = eye(size(P_bar,1));
    P_hat = (I - L*Cd)*P_bar*(I - L*Cd)' + L*Rd*L';   % Joseph form, holder seg SPD
else
    x_hat = x_bar;
    P_hat = P_bar;
end
end

== matlab function heli_q8_lab4_2020b/Kalman filter/Kf_predict ==
  data: x_hat input; P_hat input; u input; x_bar_next output; P_bar_next output; Qd parameter; Bd parameter; Ad parameter; V_s_0 parameter
function [x_bar_next, P_bar_next] = kf_predict(x_hat, P_hat, u, Qd, Bd, Ad, V_s_0)
% u = [Vs; Vd]  (Vs = kontroller FØR Vs0)
n = size(Ad, 1);
x_bar_next = zeros(n, 1);
P_bar_next = zeros(n, n);

p_hat = x_hat(1);
e_hat = x_hat(3);
Vs_eff = (u(1) + V_s_0)*cos(p_hat) - V_s_0*cos(e_hat); % torque to voltage upwards
u_eff = [Vs_eff; u(2)];

x_bar_next = Ad*x_hat + Bd*u_eff;
P_bar_next = Ad*P_hat*Ad' + Qd;
end

== matlab function heli_q8_lab4_2020b/IMU read and conversion/Low-pass filter ==
  data: y input; y_f output; fc_acc parameter
function y_f = lowpass(y, fc_acc)

persistent state
Ts = 0.002;
if isempty(state), state = y(:); end
a = exp(-2*pi*fc_acc(:)*Ts);
state = a.*state + (1 - a).*y(:);
y_f = state;
end

== matlab function heli_q8_lab4_2020b/IMU read and conversion/Low-pass filter1 ==
  data: y input; y_f output; fc_gyro parameter
function y_f = lowpass(y, fc_gyro)

persistent state
Ts = 0.002;
if isempty(state), state = y(:); end
a = exp(-2*pi*fc_gyro(:)*Ts);
state = a.*state + (1 - a).*y(:);
y_f = state;
end
